simulink model "simulink_model_advanced_closed_loop"  (R2016b)
settings: Solver=ode45  StartTime=0.0  StopTime=1  RelTol=1e-3
values from neighbouring files (symbols this model uses):
  N = 40    [extensive_example_ocp.m]    (also in minimal_example_closed_loop.m = 20; minimal_example_ocp.m = 20)
  nu = model.u.rows()    [extensive_example_ocp.m]    (also in get_pendulum_on_cart_model.m = 1; minimal_example_closed_loop.m; minimal_example_ocp.m = length(model.u))
  nx = model.x.rows()    [extensive_example_ocp.m]    (also in get_pendulum_on_cart_model.m = 4; minimal_example_closed_loop.m; minimal_example_ocp.m = length(model.x); minimal_example_sim.m = length(model.x))
  ny = nx+nu    [extensive_example_ocp.m]    (also in minimal_example_ocp.m = nx + nu)
  ny_0 = nu    [extensive_example_ocp.m]    (also in minimal_example_ocp.m)
  ny_e = nx    [extensive_example_ocp.m]    (also in minimal_example_ocp.m)
  ocp = AcadosOcp()    [extensive_example_ocp.m]    (also in minimal_example_closed_loop.m; minimal_example_ocp.m)
  U_max = 80    [minimal_example_closed_loop.m]    (also in minimal_example_ocp.m)
  x0 = [0; pi; 0; 0]    [extensive_example_ocp.m]    (also in minimal_example_closed_loop.m = x_sim(:,i); minimal_example_ocp.m; minimal_example_sim.m = [0; 1e-1; 0; 0])
settings Model: Creator=oj  LastModifiedBy=oj
settings DataIOCC: SaveFormat=StructureWithTime  ReturnWorkspaceOutputs=on
settings OptimizationCC: LifeSpan=inf
settings DebuggingCC: FcnCallInpInsideContextMsg=warning  SFExecutionAtInitializationDiag=none
settings HardwareCC: ProdBitPerSizeT=32  ProdBitPerPtrDiffT=32  ProdWordSize=32  ProdHWDeviceType=Specified
settings ModelReferenceCC: EnableRefExpFcnMdlSchedulingChecks=off
settings SFSimCC: SimUseLocalCustomCode=on
settings RTWCC: RTWUseLocalCustomCode=on

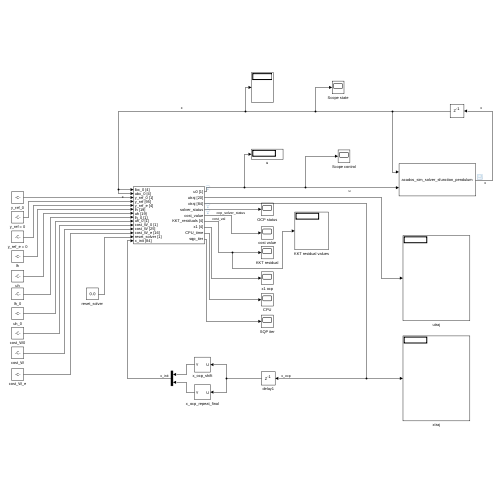
[thumbnail: Simulink's stored preview of the top-level diagram]
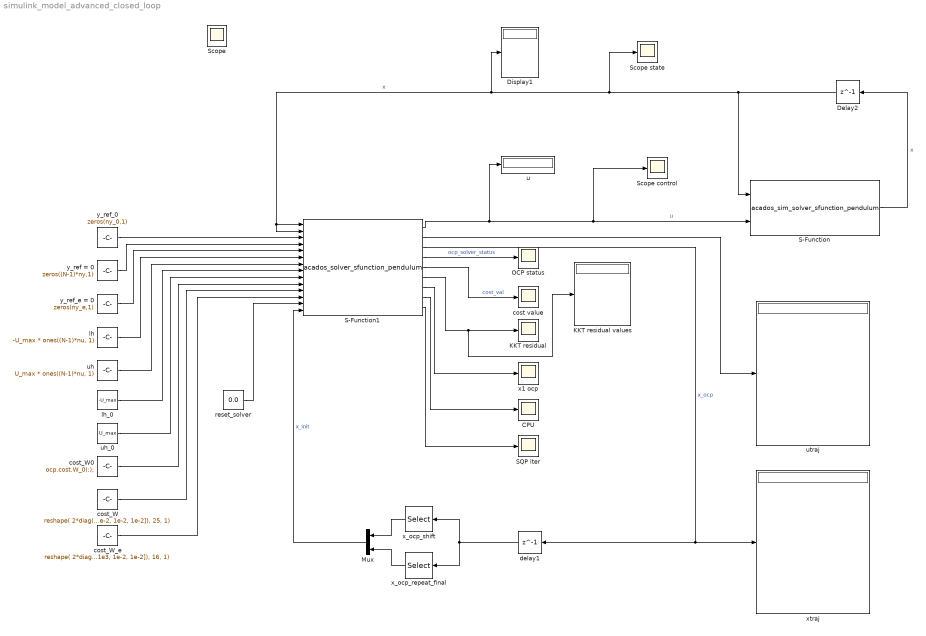
== system simulink_model_advanced_closed_loop ==
  CPU : Scope
      settings: Description=status
  Delay2 : Delay  DelayLength=1  InitialCondition=x0
  Display1 : Display
  KKT residual : Scope
      settings: Description=status
  KKT residual values : Display
  Mux : Mux  Inputs=2
  OCP status : Scope
      settings: Description=status
  S-Function : S-Function  FunctionName=acados_sim_solver_sfunction_pendulum  SFunctionDeploymentMode=off  EnableBusSupport=off
  S-Function1 : S-Function  FunctionName=acados_solver_sfunction_pendulum  SFunctionDeploymentMode=off  EnableBusSupport=off
      mask Display:
      | global sfun_input_names sfun_output_names
      | for i = 1:length(sfun_input_names)
      | 	port_label('input', i, sfun_input_names{i})
      | end
      | for i = 1:length(sfun_output_names)
      | 	port_label('output', i, sfun_output_names{i})
      | end
  SQP iter : Scope
      settings: Description=status
  Scope control : Scope
  Scope state : Scope
  cost value : Scope
      settings: Description=status
  cost_W : Constant  Value=reshape( 2*diag([1e3, 1e3, 1e-2, 1e-2, 1e-2]), 25, 1)
  cost_W0 : Constant  Value=ocp.cost.W_0(:);
  cost_W_e : Constant  Value=reshape( 2*diag([1e3, 1e3, 1e-2, 1e-2]), 16, 1)
  delay1 : Delay  DelayLength=1  InitialCondition=zeros(nx*(N+1),1)
  lh : Constant  Value=-U_max * ones((N-1)*nu, 1)
  lh_0 : Constant  Value=-U_max
  reset_solver : Constant  Value=0.0
  u : Display
  uh : Constant  Value=U_max * ones((N-1)*nu, 1)
  uh_0 : Constant  Value=U_max
  utraj : Display
  x1 ocp : Scope
      settings: Description=status
  x_ocp_repeat_final : Selector  IndexMode=Zero-based  InputPortWidth=(N+1)*nx  IndexOptions=Starting index (dialog)  Indices=N*nx  OutputSizes=nx
  x_ocp_shift : Selector  IndexMode=Zero-based  InputPortWidth=(N+1)*nx  IndexOptions=Starting index (dialog)  Indices=nx  OutputSizes=N*nx
  xtraj : Display
  y_ref = 0 : Constant  Value=zeros((N-1)*ny,1)
  y_ref_0 : Constant  Value=zeros(ny_0,1)
  y_ref_e = 0 : Constant  Value=zeros(ny_e,1)
  Scope : Scope
  wires:
  S-Function/1 -> Delay2/1  "x"
  S-Function1/4 -> OCP status/1  "ocp_solver_status"
  y_ref = 0/1 -> S-Function1/4
  y_ref_e = 0/1 -> S-Function1/5
  lh/1 -> S-Function1/6
  uh/1 -> S-Function1/7
  S-Function1/1 -> Scope control/1, S-Function/2, u/1  "u"
  Delay2/1 -> S-Function/1, Scope state/1, S-Function1/2, S-Function1/1, Display1/1  "x"
  cost_W0/1 -> S-Function1/10
  cost_W/1 -> S-Function1/11
  cost_W_e/1 -> S-Function1/12
  y_ref_0/1 -> S-Function1/3
  S-Function1/2 -> utraj/1
  x_ocp_shift/1 -> Mux/1
  delay1/1 -> x_ocp_shift/1, x_ocp_repeat_final/1
  Mux/1 -> S-Function1/14  "x_init"
  x_ocp_repeat_final/1 -> Mux/2
  S-Function1/3 -> xtraj/1, delay1/1  "x_ocp"
  reset_solver/1 -> S-Function1/13
  S-Function1/5 -> cost value/1  "cost_val"
  S-Function1/6 -> KKT residual values/1, KKT residual/1
  S-Function1/7 -> x1 ocp/1
  S-Function1/8 -> CPU/1
  S-Function1/9 -> SQP iter/1
  lh_0/1 -> S-Function1/8
  uh_0/1 -> S-Function1/9
